simulink model "simulink_eyestrain"  (R2025b)
settings: Solver=FixedStepDiscrete  StartTime=0.0  StopTime=10000  FixedStep=1  RelTol=1e-3
model workspace (MAT data in the model file):
  Distance_cm = 35
  Humidity_pct = 28
  Noise_level = 0.2
libraries: simulink x3
settings Model: Creator=User  LastModifiedBy=User

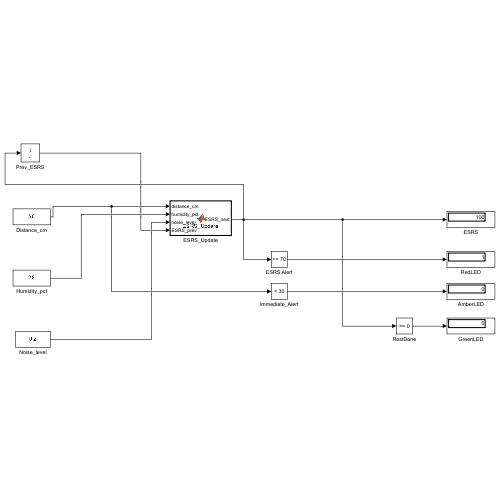
[thumbnail: Simulink's stored preview of the top-level diagram]
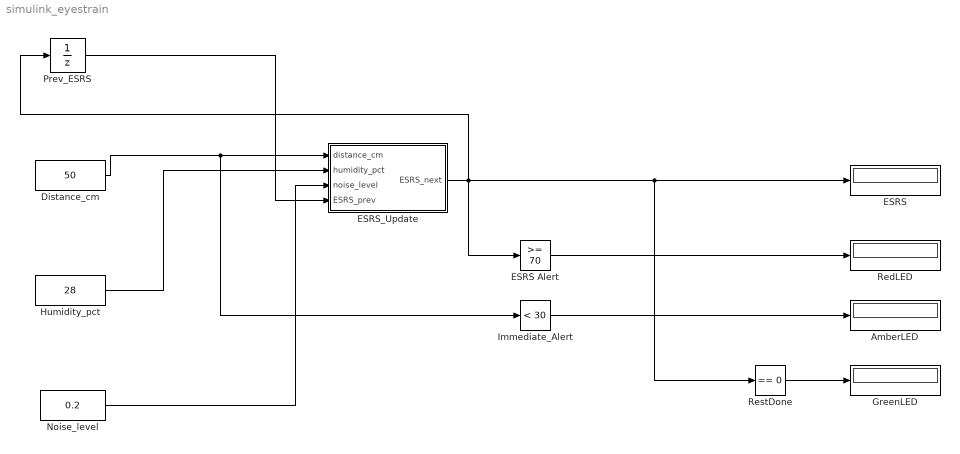
== system simulink_eyestrain ==
  AmberLED : Display
  Distance_cm : Constant  Value=50
  ESRS : Display
  ESRS Alert : simulink/Logic and Bit Operations/Compare To Constant  relop=>=  const=70  OutDataTypeStr=boolean
  ESRS_Update : MATLAB Function  TreatAsAtomicUnit=on
  GreenLED : Display
  Humidity_pct : Constant  Value=28
  Immediate_Alert : simulink/Logic and Bit Operations/Compare To Constant  relop=<  const=30  OutDataTypeStr=boolean
  Noise_level : Constant  Value=0.2
  Prev_ESRS : UnitDelay  SampleTime=-1  HasFrameUpgradeWarning=on
  RedLED : Display
  RestDone : simulink/Logic and Bit Operations/Compare To Constant  relop===  const=0  OutDataTypeStr=boolean
  wires:
  Distance_cm/1 -> Immediate_Alert/1, ESRS_Update/1(distance_cm)
  Humidity_pct/1 -> ESRS_Update/2(humidity_pct)
  Prev_ESRS/1 -> ESRS_Update/4(ESRS_prev)
  ESRS_Update/1(ESRS_next) -> Prev_ESRS/1, ESRS/1, RestDone/1, ESRS Alert/1
  Noise_level/1 -> ESRS_Update/3(noise_level)
  Immediate_Alert/1 -> AmberLED/1
  RestDone/1 -> GreenLED/1
  ESRS Alert/1 -> RedLED/1

== matlab function simulink_eyestrain/ESRS_Update ==
  data: distance_cm input; ESRS_next output; humidity_pct input; noise_level input; ESRS_prev input
function ESRS_next = ESRS_Update(distance_cm, humidity_pct, noise_level, ESRS_prev)
%#codegen

dryHumidityThreshold = 40;
highNoiseThreshold = 0.6;

riskMin = 0;
riskMax = 100;

rate_under30 = 15.0;
rate_30_40   = 4.5;
rate_40_60   = 2.0;
rate_60_100  = 0.1;
rate_over100 = -6.0;

dryMultiplier = 1.30;
noiseMultiplier = 1.20;

dt = 1; % seconds

isDry = humidity_pct < dryHumidityThreshold;
isNoisy = noise_level >= highNoiseThreshold;

if distance_cm < 30
    deltaPerMin = rate_under30;
elseif distance_cm < 40
    deltaPerMin = rate_30_40;
elseif distance_cm < 60
    deltaPerMin = rate_40_60;
elseif distance_cm <= 100
    deltaPerMin = rate_60_100;
else
    deltaPerMin = rate_over100;
end

if distance_cm < 60
    if isDry
        deltaPerMin = deltaPerMin * dryMultiplier;
    end
    if isNoisy
        deltaPerMin = deltaPerMin * noiseMultiplier;
    end
end

delta = deltaPerMin * (dt / 60);
ESRS_next = ESRS_prev + delta;

if ESRS_next > riskMax
    ESRS_next = riskMax;
elseif ESRS_next < riskMin
    ESRS_next = riskMin;
end
